simulink model "Buck_Closed_Loop"  (R2023b)
settings: Solver=VariableStepAuto  StartTime=0.0  StopTime=0.1  RelTol=1e-3
libraries: spsSeriesRLCBranchLib x9, spsIdealSwitchLib x3, spsVoltageMeasurementLib x2, slpidlib x2, spsCurrentMeasurementLib x1, spsDCVoltageSourceLib x1, spsDiodeLib x1, spsMosfetLib x1, spspowerguiLib x1, simulink x1
settings Model: Creator=Qu  LastModifiedBy=Qu

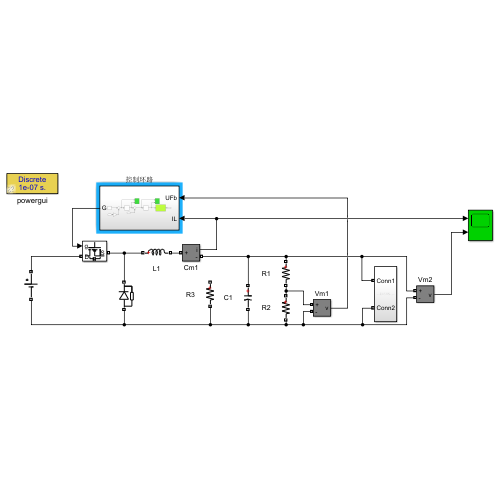
[thumbnail: Simulink's stored preview of the top-level diagram]
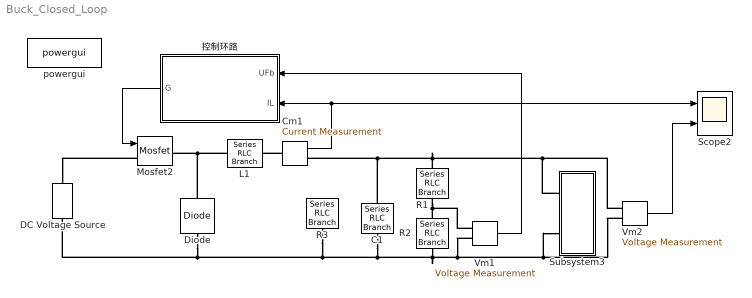
== system Buck_Closed_Loop ==
  C1 : spsSeriesRLCBranchLib/Series RLC Branch  LConnTagsString=__new0  RConnTagsString=__new0  BranchType=C  Resistance=0.1  Inductance=0  SetiL0=off  InitialCurrent=0  Capacitance=1e-4  Setx0=off  InitialVoltage=310  Measurements=None
  Cm1 : spsCurrentMeasurementLib/Current Measurement  PhasorSimulation=off  OutputType=Complex  PSBequivalent=0
  DC Voltage Source : spsDCVoltageSourceLib/DC Voltage Source  Amplitude=220  Measurements=None
  Diode : spsDiodeLib/Diode  Ron=0.001  Lon=0  Vf=1  IC=0  UseSnubber=0  Rs=47  Cs=1e-9  Measurements=off
  L1 : spsSeriesRLCBranchLib/Series RLC Branch  LConnTagsString=__new0  RConnTagsString=__new0  BranchType=L  Resistance=0.01  Inductance=8e-4  SetiL0=off  InitialCurrent=0  Capacitance=inf  Setx0=off  InitialVoltage=0  Measurements=None
  Mosfet2 : spsMosfetLib/Mosfet  Ron=0.05  Lon=0  Rd=0.01  Vfd=1  IC=0  Rs=1e5  Cs=inf  Measurements=off
  R1 : spsSeriesRLCBranchLib/Series RLC Branch  LConnTagsString=__new0  RConnTagsString=__new0  BranchType=R  Resistance=47e3  Inductance=0  SetiL0=off  InitialCurrent=0  Capacitance=4e-3  Setx0=on  InitialVoltage=310  Measurements=None
  R2 : spsSeriesRLCBranchLib/Series RLC Branch  LConnTagsString=__new0  RConnTagsString=__new0  BranchType=R  Resistance=1e3  Inductance=0  SetiL0=off  InitialCurrent=0  Capacitance=4e-3  Setx0=on  InitialVoltage=310  Measurements=None
  R3 : spsSeriesRLCBranchLib/Series RLC Branch  LConnTagsString=__new0  RConnTagsString=__new0  BranchType=R  Resistance=100  Inductance=0  SetiL0=off  InitialCurrent=0  Capacitance=4e-3  Setx0=on  InitialVoltage=310  Measurements=None
  Scope2 : Scope  NumInputPorts=2
  Subsystem3 : Subsystem
      settings: PortSchema="{\"entries\":[{\"content\":{\"sides\":[{\"content\":{},\"type\":\"ConnectorPlacement.EquallySpacedRectSide\",\"uuid\":\"d898510c-3808-4901-b4c2-b237505f3f1a\"},{\"content\":{\"side\":\"RIGHT\"},\"type\":\"ConnectorPlacement.EquallySpacedRectSide\",\"uuid\":\"23020826-9030-48c4-aa04-efdffa804e53\"},{\"content\":{\"connectorIds\":[\"LConn1\",\"LConn2\"],\"side\":\"TOP\"},\"type\":\"ConnectorPlacement.EquallySpacedRectSide\",\"uuid\":\"14d0c90e-d12e-4876-8eae-a6da1cc835ce\"}]},\"type\":\"ConnectorPlacement.EquallySpacedConnector\",\"uuid\":\"078ec9a7-4da9-4ce0-9ae3-53c66093e52b\"}],\"packageUris\":[\"http://schema.mathworks.com/mf0/Connector/R2020b\"],\"version\":\"1.0\"}"
  Vm1 : spsVoltageMeasurementLib/Voltage Measurement  PhasorSimulation=off  OutputType=Complex  PSBequivalent=0
  Vm2 : spsVoltageMeasurementLib/Voltage Measurement  PhasorSimulation=off  OutputType=Complex  PSBequivalent=0
  powergui : spspowerguiLib/powergui  SimulationMode=Discrete  SampleTime=1e-7  frequency=60  Iterations=50  frequencyindice=0  Pbase=100e6  ErrMax=1e-4  UnitsV=kV  UnitsW=MW  buscounter=0  FunctionMessages=off  echomessages=off  EnableUseOfTLC=off  CurrentSourceSwitches=off  DisableSnubberDevices=off  DisableRonSwitches=off  DisableVfSwitches=off  DisplayEquations=off  AutomaticDiscreteSolvers=off  SolverType=Tustin/Backward Euler (TBE)  Interpol=off  ExternalGateDelay=off  methode=off  Ts=0  x0status=blocks  SPID=off  SwTol=0  HookPort=off  NonlinearTolerance=1e-4  nMaxIteration=100  ContinueOnMaxIteration=off  RestoreLinks=warning  ResistiveCurrentMeasurement=off  Frange=[0:2:500]  Ylog=off  Xlog=on  ShowGrid=off  save=off  variable=ZData  structure=QQQQQ  ZoomFFT=off  StartTime=0.5  cycles=15  DisplayStyle=1  fundamental=50  FreqAxis=off  MaxFrequency=1000  frequencyindicesteady=1  RmsSteady=1  display=off
  控制环路 : Subsystem
      settings: PortSchema="{\"entries\":[{\"content\":{\"sides\":[{\"content\":{\"connectorIds\":[\"Out1\"]},\"type\":\"ConnectorPlacement.EquallySpacedRectSide\",\"uuid\":\"e7b426f2-4b92-4d8e-bbef-a0ce76254dbe\"},{\"content\":{\"connectorIds\":[\"In1\",\"In2\"],\"side\":\"RIGHT\"},\"type\":\"ConnectorPlacement.EquallySpacedRectSide\",\"uuid\":\"4156ee22-87ce-4752-802f-1538deb6fdc0\"},{\"content\":{\"side\":\"TOP\"},\"type\":\"ConnectorPlacement.EquallySpacedRectSide\",\"uuid\":\"2109ac6d-f656-40e1-b9b4-63dfb0a9bde6\"}]},\"type\":\"ConnectorPlacement.EquallySpacedConnector\",\"uuid\":\"abd2b871-34eb-4c5b-8139-0f5dd8971ed6\"}],\"packageUris\":[\"http://schema.mathworks.com/mf0/Connector/R2020b\"],\"version\":\"1.0\"}"
  wires:
  控制环路/1(G) -> Mosfet2/1
  Cm1/1 -> 控制环路/2(IL), Scope2/1
  Vm1/1 -> 控制环路/1(UFb)
  Vm2/1 -> Scope2/2
  connections:
  Diode/RConn1 -- Mosfet2/RConn1 -- L1/LConn1
  Mosfet2/LConn1 -- DC Voltage Source/RConn1
  Diode/LConn1 -- Vm2/LConn2 -- Subsystem3/LConn2 -- Vm1/LConn2 -- R2/RConn1 -- C1/RConn1 -- R3/RConn1 -- DC Voltage Source/LConn1
  Cm1/LConn1 -- L1/RConn1
  C1/LConn1 -- Subsystem3/LConn1 -- Vm2/LConn1 -- R1/LConn1 -- Cm1/RConn1
  R2/LConn1 -- Vm1/LConn1 -- R1/RConn1

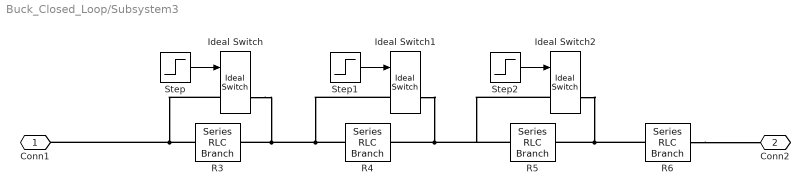
== system Buck_Closed_Loop/Subsystem3 ==
  Ideal Switch : spsIdealSwitchLib/Ideal Switch  Ron=0.0000000001  Lon=0  IC=0  Rs=1e5  Cs=inf  Measurements=on
  Ideal Switch1 : spsIdealSwitchLib/Ideal Switch  Ron=0.0000000001  Lon=0  IC=0  Rs=1e5  Cs=inf  Measurements=on
  Ideal Switch2 : spsIdealSwitchLib/Ideal Switch  Ron=0.0000000001  Lon=0  IC=0  Rs=1e5  Cs=inf  Measurements=on
  R3 : spsSeriesRLCBranchLib/Series RLC Branch  LConnTagsString=__new0  RConnTagsString=__new0  BranchType=R  Resistance=50  Inductance=1e-3  SetiL0=off  InitialCurrent=0  Capacitance=1e-6  Setx0=off  InitialVoltage=0  Measurements=None
  R4 : spsSeriesRLCBranchLib/Series RLC Branch  LConnTagsString=__new0  RConnTagsString=__new0  BranchType=R  Resistance=30  Inductance=1e-3  SetiL0=off  InitialCurrent=0  Capacitance=1e-6  Setx0=off  InitialVoltage=0  Measurements=None
  R5 : spsSeriesRLCBranchLib/Series RLC Branch  LConnTagsString=__new0  RConnTagsString=__new0  BranchType=R  Resistance=10  Inductance=1e-3  SetiL0=off  InitialCurrent=0  Capacitance=1e-6  Setx0=off  InitialVoltage=0  Measurements=None
  R6 : spsSeriesRLCBranchLib/Series RLC Branch  LConnTagsString=__new0  RConnTagsString=__new0  BranchType=R  Resistance=10  Inductance=1e-3  SetiL0=off  InitialCurrent=0  Capacitance=1e-6  Setx0=off  InitialVoltage=0  Measurements=None
  Step : Step  Time=0.03  SampleTime=0
  Step1 : Step  Time=0.05  SampleTime=0
  Step2 : Step  Time=0.07  SampleTime=0
  Conn1 : PMIOPort  Side=Left
  Conn2 : PMIOPort  Port=2  Side=Left
  wires:
  Step1/1 -> Ideal Switch1/1
  Step2/1 -> Ideal Switch2/1
  Step/1 -> Ideal Switch/1
  connections:
  Ideal Switch1/RConn1 -- R4/RConn1 -- R5/LConn1 -- Ideal Switch2/LConn1
  R4/LConn1 -- R3/RConn1 -- Ideal Switch/RConn1 -- Ideal Switch1/LConn1
  Ideal Switch/LConn1 -- R3/LConn1 -- Conn1/RConn1
  R6/LConn1 -- R5/RConn1 -- Ideal Switch2/RConn1
  R6/RConn1 -- Conn2/RConn1

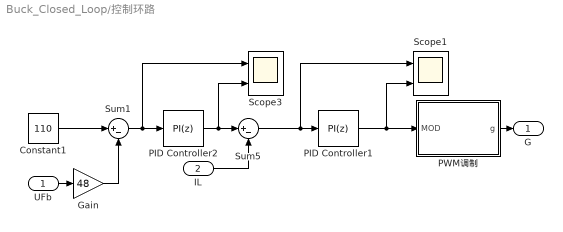
== system Buck_Closed_Loop/控制环路 ==
  UFb : Inport
  IL : Inport  Port=2
  Constant1 : Constant  Value=110
  Gain : Gain  Gain=48
  PID Controller1 : slpidlib/PID Controller  Controller=PI  Form=Parallel  TimeDomain=Discrete-time  UseExternalTs=off  SampleTime=1/100000  IntegratorMethod=Forward Euler  FilterMethod=Forward Euler  ControllerParametersSource=internal  P=0.1  I=100  UseKiTs=off  D=0.001  N=100  UseFilter=on  TunerSelectOption=Transfer Function Based (PID Tuner App)  InitialConditionSource=internal  InitialConditionForIntegrator=0  InitialConditionForFilter=0  DifferentiatorICPrevScaledInput=0  ExternalReset=none  TrackingMode=off  Kt=1  LimitOutput=on  SatLimitsSource=internal  UpperSaturationLimit=1  LowerSaturationLimit=0  LinearizeAsGain=on  AntiWindupMode=clamping  Kb=1  LimitIntegrator=on  UpperIntegratorSaturationLimit=1  LowerIntegratorSaturationLimit=0  POutMin=[]  POutMax=[]  IOutMin=[]  IOutMax=[]  DOutMin=[]  DOutMax=[]  NOutMin=[]  NOutMax=[]  SumOutMin=[]  SumOutMax=[]  SaturationOutMin=[]  SaturationOutMax=[]  PParamMin=[]  PParamMax=[]  IParamMin=[]  IParamMax=[]  DParamMin=[]  DParamMax=[]  NParamMin=[]  NParamMax=[]  KbParamMin=[]  KbParamMax=[]  KtParamMin=[]  KtParamMax=[]  KbOutMin=[]  KbOutMax=[]  KtOutMin=[]  KtOutMax=[]  IntegratorOutMin=[]  IntegratorOutMax=[]  FilterOutMin=[]  FilterOutMax=[]  SumI1OutMin=[]  SumI1OutMax=[]  SumI2OutMin=[]  SumI2OutMax=[]  SumI3OutMin=[]  SumI3OutMax=[]  SumI4OutMin=[]  SumI4OutMax=[]  SumDOutMin=[]  SumDOutMax=[]  DifferentiatorOutMin=[]  DifferentiatorOutMax=[]  FilterDiffOutCoefMin=[]  FilterDiffOutCoefMax=[]  ReciprocalOutMin=[]  ReciprocalOutMax=[]  SumDenOutMin=[]  SumDenOutMax=[]  SumNumOutMin=[]  SumNumOutMax=[]  DivideOutMin=[]  DivideOutMax=[]  UdiffTsProdOutMin=[]  UdiffTsProdOutMax=[]  NTsProdOutMin=[]  NTsProdOutMax=[]  UintegralTsProdOutMin=[]  UintegralTsProdOutMax=[]  UngainTsProdOutMin=[]  UngainTsProdOutMax=[]  ClampingZeroOutDataTypeStr=Inherit: Inherit via back propagation  ClampingZeroOutMin=[]  ClampingZeroOutMax=[]  FilterDenConstantOutDataTypeStr=Inherit: Inherit via back propagation  FilterDenConstantOutMin=[]  FilterDenConstantOutMax=[]  PCopyOutDataTypeStr=Inherit: Inherit via back propagation  PCopyOutMin=[]  PCopyOutMax=[]  NCopyOutDataTypeStr=Inherit: Inherit via back propagation  NCopyOutMin=[]  NCopyOutMax=[]  IntegratorContinuousStateAttributes=''  IntegratorStateMustResolveToSignalObject=off  IntegratorRTWStateStorageClass=Auto  FilterContinuousStateAttributes=''  FilterStateMustResolveToSignalObject=off  FilterRTWStateStorageClass=Auto  ParallelPVariant=InternalParameters  IdealPVariant=Disabled  IVariant=InternalParameters  DVariant=Disabled  IntegratorVariant=Discrete  SatVariant=Enabled  AWVariant=DiscClampingParallel  PCopyVariant=Disabled  TRVariant=Disabled  FdbkBlocksVariant=Forward  IdealPFdbkVariant=Disabled  SatFdbkVariant=Disabled  DerivativeFilterVariant=Disabled  NVariant=Disabled  NCopyVariant=Disabled_SignalSpec  FilterICVariant=Disabled  IntegratorICVariant=InternalICs  ExternalResetVariant=Disabled  TRSumVariant=Passthrough  SumFdbkVariant=Disabled  SumVariant=Sum_PI  TsampFilterVariant=InternalTs  TsampNgainVariant=Passthrough  TsampIntegralVariant=Disabled_SignalSpec  ExternalSaturationOutDataTypeStr=Inherit: Same as second input
  PID Controller2 : slpidlib/PID Controller  Controller=PI  Form=Parallel  TimeDomain=Discrete-time  UseExternalTs=off  SampleTime=1/100000  IntegratorMethod=Forward Euler  FilterMethod=Forward Euler  ControllerParametersSource=internal  P=9  I=60000  UseKiTs=off  D=0.001  N=100  UseFilter=on  TunerSelectOption=Transfer Function Based (PID Tuner App)  InitialConditionSource=internal  InitialConditionForIntegrator=0  InitialConditionForFilter=0  DifferentiatorICPrevScaledInput=0  ExternalReset=none  TrackingMode=off  Kt=1  LimitOutput=on  SatLimitsSource=internal  UpperSaturationLimit=12  LowerSaturationLimit=0  LinearizeAsGain=on  AntiWindupMode=clamping  Kb=1  LimitIntegrator=on  UpperIntegratorSaturationLimit=12  LowerIntegratorSaturationLimit=0  POutMin=[]  POutMax=[]  IOutMin=[]  IOutMax=[]  DOutMin=[]  DOutMax=[]  NOutMin=[]  NOutMax=[]  SumOutMin=[]  SumOutMax=[]  SaturationOutMin=[]  SaturationOutMax=[]  PParamMin=[]  PParamMax=[]  IParamMin=[]  IParamMax=[]  DParamMin=[]  DParamMax=[]  NParamMin=[]  NParamMax=[]  KbParamMin=[]  KbParamMax=[]  KtParamMin=[]  KtParamMax=[]  KbOutMin=[]  KbOutMax=[]  KtOutMin=[]  KtOutMax=[]  IntegratorOutMin=[]  IntegratorOutMax=[]  FilterOutMin=[]  FilterOutMax=[]  SumI1OutMin=[]  SumI1OutMax=[]  SumI2OutMin=[]  SumI2OutMax=[]  SumI3OutMin=[]  SumI3OutMax=[]  SumI4OutMin=[]  SumI4OutMax=[]  SumDOutMin=[]  SumDOutMax=[]  DifferentiatorOutMin=[]  DifferentiatorOutMax=[]  FilterDiffOutCoefMin=[]  FilterDiffOutCoefMax=[]  ReciprocalOutMin=[]  ReciprocalOutMax=[]  SumDenOutMin=[]  SumDenOutMax=[]  SumNumOutMin=[]  SumNumOutMax=[]  DivideOutMin=[]  DivideOutMax=[]  UdiffTsProdOutMin=[]  UdiffTsProdOutMax=[]  NTsProdOutMin=[]  NTsProdOutMax=[]  UintegralTsProdOutMin=[]  UintegralTsProdOutMax=[]  UngainTsProdOutMin=[]  UngainTsProdOutMax=[]  ClampingZeroOutDataTypeStr=Inherit: Inherit via back propagation  ClampingZeroOutMin=[]  ClampingZeroOutMax=[]  FilterDenConstantOutDataTypeStr=Inherit: Inherit via back propagation  FilterDenConstantOutMin=[]  FilterDenConstantOutMax=[]  PCopyOutDataTypeStr=Inherit: Inherit via back propagation  PCopyOutMin=[]  PCopyOutMax=[]  NCopyOutDataTypeStr=Inherit: Inherit via back propagation  NCopyOutMin=[]  NCopyOutMax=[]  IntegratorContinuousStateAttributes=''  IntegratorStateMustResolveToSignalObject=off  IntegratorRTWStateStorageClass=Auto  FilterContinuousStateAttributes=''  FilterStateMustResolveToSignalObject=off  FilterRTWStateStorageClass=Auto  ParallelPVariant=InternalParameters  IdealPVariant=Disabled  IVariant=InternalParameters  DVariant=Disabled  IntegratorVariant=Discrete  SatVariant=Enabled  AWVariant=DiscClampingParallel  PCopyVariant=Disabled  TRVariant=Disabled  FdbkBlocksVariant=Forward  IdealPFdbkVariant=Disabled  SatFdbkVariant=Disabled  DerivativeFilterVariant=Disabled  NVariant=Disabled  NCopyVariant=Disabled_SignalSpec  FilterICVariant=Disabled  IntegratorICVariant=InternalICs  ExternalResetVariant=Disabled  TRSumVariant=Passthrough  SumFdbkVariant=Disabled  SumVariant=Sum_PI  TsampFilterVariant=InternalTs  TsampNgainVariant=Passthrough  TsampIntegralVariant=Disabled_SignalSpec  ExternalSaturationOutDataTypeStr=Inherit: Same as second input
  PWM调制 : Subsystem
  Scope1 : Scope  NumInputPorts=2
  Scope3 : Scope  NumInputPorts=2
  Sum1 : Sum  Inputs=|+-
  Sum5 : Sum  Inputs=|+-
  G : Outport
  wires:
  Sum5/1 -> Scope1/1, PID Controller1/1
  Sum1/1 -> Scope3/1, PID Controller2/1
  PID Controller2/1 -> Scope3/2, Sum5/1
  Constant1/1 -> Sum1/1
  IL/1 -> Sum5/2
  UFb/1 -> Gain/1
  Gain/1 -> Sum1/2
  PID Controller1/1 -> PWM调制/1(MOD), Scope1/2
  PWM调制/1(g) -> G/1

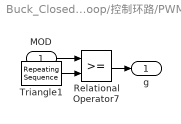
== system Buck_Closed_Loop/控制环路/PWM调制 ==
  MOD : Inport
  Relational Operator7 : RelationalOperator  OutDataTypeStr=boolean  InputSameDT=off
  Triangle1 : simulink/Sources/Repeating Sequence  rep_seq_t=[0 1/100000/2 1/100000]  rep_seq_y=[0 1 0]
  g : Outport
  wires:
  Relational Operator7/1 -> g/1
  Triangle1/1 -> Relational Operator7/2
  MOD/1 -> Relational Operator7/1
